simulink model "PositionControl"  (R2023b)
settings: Solver=FixedStepAuto  StartTime=0.0  StopTime=100.0  FixedStep=Ts  RelTol=1e-3
values from neighbouring files (symbols this model uses):
  refx = refs(i, 1)    [CompararControladores.m]    (also in GenerarDatosControl.m = 10*rand - 5; RunPositionControl.m = 2)
  refy = refs(i, 2)    [CompararControladores.m]    (also in GenerarDatosControl.m = 10*rand - 5; RunPositionControl.m = 2)
undefined symbols (not defined in the file or in its folder): DiscIntNeverNeededParam
settings Model: Creator=perez  LastModifiedBy=perez
settings DataIOCC: ReturnWorkspaceOutputs=off

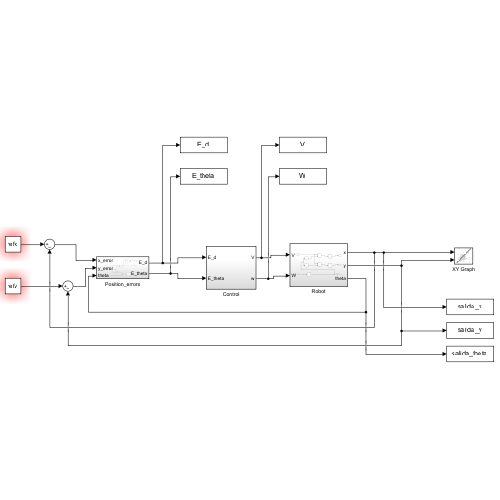
[thumbnail: Simulink's stored preview of the top-level diagram]
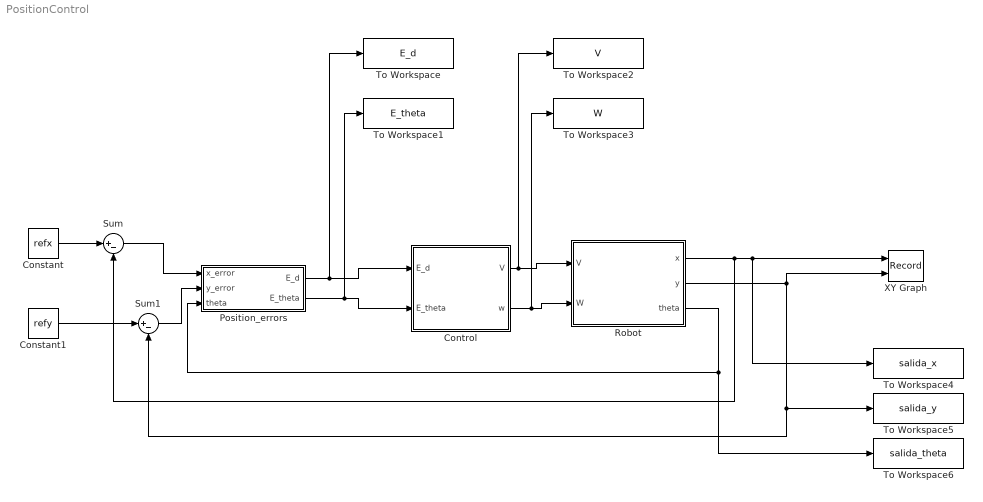
== system PositionControl ==
  Constant : Constant  Value=refx
  Constant1 : Constant  Value=refy
  Control : Subsystem
  Position_errors : Subsystem
  Robot : Subsystem
  Sum : Sum  Inputs=|+-
  Sum1 : Sum  Inputs=|+-
  To Workspace : ToWorkspace  VariableName=E_d  SaveFormat=Structure With Time  SampleTime=-1
  To Workspace1 : ToWorkspace  VariableName=E_theta  SaveFormat=Structure With Time  SampleTime=-1
  To Workspace2 : ToWorkspace  VariableName=V  SaveFormat=Structure With Time  SampleTime=-1
  To Workspace3 : ToWorkspace  VariableName=W  SaveFormat=Structure With Time  SampleTime=-1
  To Workspace4 : ToWorkspace  VariableName=salida_x  SaveFormat=Structure With Time  SampleTime=-1
  To Workspace5 : ToWorkspace  VariableName=salida_y  SaveFormat=Structure With Time  SampleTime=-1
  To Workspace6 : ToWorkspace  VariableName=salida_theta  SaveFormat=Structure With Time  SampleTime=-1
  XY Graph : Record  FileSettingsInternal="{\"entries\":[{\"content\":{\"excelSettings\":{\"content\":{},\"type\":\"Streamout.ExcelSettings\"}},\"type\":\"Streamout.FileSettingStorage\",\"uuid\":\"\"}],\"packageUris\":[\"http:\\/\\/schema.mathworks.com\\/mf0\\/streamout_blocks\\/R2020a\"],\"version\":\"1.0\"}"  Layout=[1 1]  SignalsInternal="{\"entries\":[{\"content\":{\"signals\":[{\"content\":{\"blockPath\":[],\"dimensions\":[1],\"domain\":\"\",\"lineColor\":\"#a2142f\",\"plots\":[ 1 ],\"port\":1,\"signalID\":1,\"signalName\":\"XY Graph:1\"},\"type\":\"RecordBlkView.Signal\",\"uuid\":\"\"},{\"content\":{\"blockPath\":[],\"dimensions\":[1],\"domain\":\"\",\"lineColor\":\"#139fff\",\"plots\":[ 1 ],\"port\":2,\"signalID\":2,\"signalName\":\"XY Graph:2\"},\"type\":\"RecordBlkView.Signal\",\"uuid\":\"\"}]},\"type\":\"RecordBlkView.InputSignals\",\"uuid\":\"\"}],\"packageUris\":[\"http:\\/\\/schema.mathworks.com\\/mf0\\/streamout_blocks\\/R2020a\"],\"version\":\"1.0\"}"  VisualizationBindings="{\"xyplotplugin\":{\"info\":[{\"series\":[{\"bindingParametersList\":[{\"parameter\":\"X-Axis\",\"signalID\":1,\"signalName\":\"XY Graph:1\"},{\"parameter\":\"Y-Axis\",\"signalID\":2,\"signalName\":\"XY Graph:2\"}],\"seriesID\":0}],\"subplotID\":1}]}}"  CompatibilityTag=XY
  wires:
  Constant/1 -> Sum/1
  Sum/1 -> Position_errors/1(x_error)
  Sum1/1 -> Position_errors/2(y_error)
  Position_errors/1(E_d) -> Control/1(E_d), To Workspace/1
  Position_errors/2(E_theta) -> To Workspace1/1, Control/2(E_theta)
  Control/1(V) -> To Workspace2/1, Robot/1(V)
  Control/2(w) -> To Workspace3/1, Robot/2(W)
  Robot/1(x) -> Sum/2, To Workspace4/1, XY Graph/1
  Robot/2(y) -> To Workspace5/1, Sum1/2, XY Graph/2
  Robot/3(theta) -> To Workspace6/1, Position_errors/3(theta)
  Constant1/1 -> Sum1/1

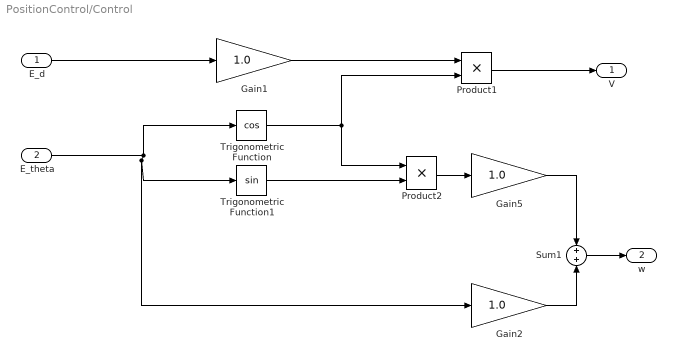
== system PositionControl/Control ==
  E_d : Inport
  E_theta : Inport  Port=2
  Gain1 : Gain  Gain=1.0
  Gain2 : Gain  Gain=1.0
  Gain5 : Gain  Gain=1.0
  Product1 : Product
  Product2 : Product
  Sum1 : Sum
  Trigonometric Function : Trigonometry  Operator=cos
  Trigonometric Function1 : Trigonometry
  V : Outport  VectorParamsAs1DForOutWhenUnconnected=off
  w : Outport  Port=2  VectorParamsAs1DForOutWhenUnconnected=off
  wires:
  E_theta/1 -> Trigonometric Function/1, Trigonometric Function1/1, Gain2/1
  E_d/1 -> Gain1/1
  Trigonometric Function/1 -> Product1/2, Product2/1
  Product1/1 -> V/1
  Trigonometric Function1/1 -> Product2/2
  Product2/1 -> Gain5/1
  Gain1/1 -> Product1/1
  Gain5/1 -> Sum1/1
  Gain2/1 -> Sum1/2
  Sum1/1 -> w/1

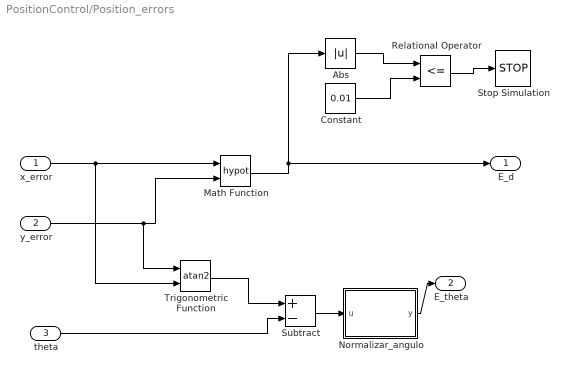
== system PositionControl/Position_errors ==
  x_error : Inport
  y_error : Inport  Port=2
  theta : Inport  Port=3
  Abs : Abs  SaturateOnIntegerOverflow=off
  Constant : Constant  Value=0.01
  Math Function : Math  Operator=hypot
  Normalizar_angulo : MATLAB Function  TreatAsAtomicUnit=on
  Relational Operator : RelationalOperator  Operator=<=  OutDataTypeStr=boolean  RndMeth=Simplest  InputSameDT=off
  Stop Simulation : Stop
  Subtract : Sum  Inputs=+-
  Trigonometric Function : Trigonometry  Operator=atan2
  E_d : Outport
  E_theta : Outport  Port=2
  wires:
  x_error/1 -> Trigonometric Function/2, Math Function/1
  y_error/1 -> Trigonometric Function/1, Math Function/2
  Trigonometric Function/1 -> Subtract/1
  theta/1 -> Subtract/2
  Subtract/1 -> Normalizar_angulo/1(u)
  Normalizar_angulo/1(y) -> E_theta/1
  Abs/1 -> Relational Operator/1
  Constant/1 -> Relational Operator/2
  Math Function/1 -> E_d/1, Abs/1
  Relational Operator/1 -> Stop Simulation/1

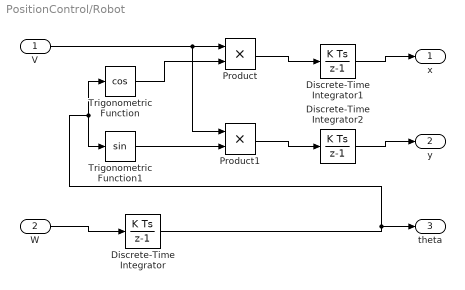
== system PositionControl/Robot ==
  V : Inport
  W : Inport  Port=2
  Discrete-Time Integrator : DiscreteIntegrator  SampleTime=-1  ICPrevOutput=DiscIntNeverNeededParam  ICPrevScaledInput=DiscIntNeverNeededParam
  Discrete-Time Integrator1 : DiscreteIntegrator  SampleTime=-1  ICPrevOutput=DiscIntNeverNeededParam  ICPrevScaledInput=DiscIntNeverNeededParam
  Discrete-Time Integrator2 : DiscreteIntegrator  SampleTime=-1  ICPrevOutput=DiscIntNeverNeededParam  ICPrevScaledInput=DiscIntNeverNeededParam
  Product : Product
  Product1 : Product
  Trigonometric Function : Trigonometry  Operator=cos
  Trigonometric Function1 : Trigonometry
  x : Outport
  y : Outport  Port=2
  theta : Outport  Port=3
  wires:
  Trigonometric Function1/1 -> Product1/2
  Discrete-Time Integrator2/1 -> y/1
  Discrete-Time Integrator1/1 -> x/1
  Product/1 -> Discrete-Time Integrator1/1
  Product1/1 -> Discrete-Time Integrator2/1
  V/1 -> Product1/1, Product/1
  Discrete-Time Integrator/1 -> Trigonometric Function1/1, Trigonometric Function/1, theta/1
  Trigonometric Function/1 -> Product/2
  W/1 -> Discrete-Time Integrator/1

== matlab function PositionControl/Position_errors/Normalizar_angulo ==
  data: u input; y output
function y = fcn(u)
% Lleva el ángulo u (rad) a su equivalente en [-pi, pi):
% +pi pasa el intervalo a [0, 2pi), mod quita las vueltas completas
% (también con u negativo) y -pi lo devuelve al intervalo original
y = mod(u + pi, 2*pi) - pi;
